simulink model "FMT_G1_ExecutionCore"  (R2026b)
settings: Solver=FixedStepDiscrete  StopTime=2  FixedStep=0.0005
model workspace (MAT data in the model file):
  stop_ticks = 4000
settings Model: Creator=26718  LastModifiedBy=26718

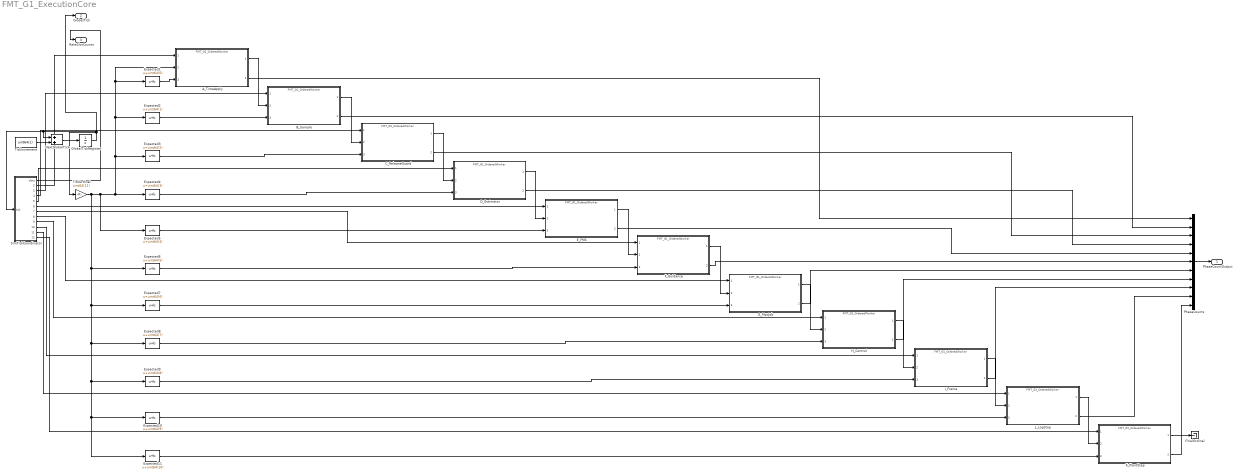
== system FMT_G1_ExecutionCore ==
  A_TimeApply : ModelReference  ModelNameDialog=FMT_G1_OrderedWorker  SimulationMode=Normal  ScheduleRates=on  ModelReferenceVersion=1.2
  B_Sample : ModelReference  ModelNameDialog=FMT_G1_OrderedWorker  SimulationMode=Normal  ScheduleRates=on  ModelReferenceVersion=1.2
  C_ReleaseGuard : ModelReference  ModelNameDialog=FMT_G1_OrderedWorker  SimulationMode=Normal  ScheduleRates=on  ModelReferenceVersion=1.2
  D_Estimator : ModelReference  ModelNameDialog=FMT_G1_OrderedWorker  SimulationMode=Normal  ScheduleRates=on  ModelReferenceVersion=1.2
  E_FMS : ModelReference  ModelNameDialog=FMT_G1_OrderedWorker  SimulationMode=Normal  ScheduleRates=on  ModelReferenceVersion=1.2
  Expected1 : Bias  Bias=uint64(0)  SaturateOnIntegerOverflow=off
  Expected10 : Bias  Bias=uint64(9)  SaturateOnIntegerOverflow=off
  Expected11 : Bias  Bias=uint64(10)  SaturateOnIntegerOverflow=off
  Expected2 : Bias  Bias=uint64(1)  SaturateOnIntegerOverflow=off
  Expected3 : Bias  Bias=uint64(2)  SaturateOnIntegerOverflow=off
  Expected4 : Bias  Bias=uint64(3)  SaturateOnIntegerOverflow=off
  Expected5 : Bias  Bias=uint64(4)  SaturateOnIntegerOverflow=off
  Expected6 : Bias  Bias=uint64(5)  SaturateOnIntegerOverflow=off
  Expected7 : Bias  Bias=uint64(6)  SaturateOnIntegerOverflow=off
  Expected8 : Bias  Bias=uint64(7)  SaturateOnIntegerOverflow=off
  Expected9 : Bias  Bias=uint64(8)  SaturateOnIntegerOverflow=off
  F_Guidance : ModelReference  ModelNameDialog=FMT_G1_OrderedWorker  SimulationMode=Normal  ScheduleRates=on  ModelReferenceVersion=1.2
  FinalOrdinal : Terminator
  G_MpcJob : ModelReference  ModelNameDialog=FMT_G1_OrderedWorker  SimulationMode=Normal  ScheduleRates=on  ModelReferenceVersion=1.2
  GlobalTickRegister : UnitDelay  InitialCondition=uint64(0)  SampleTime=0.0005
  H_Control : ModelReference  ModelNameDialog=FMT_G1_OrderedWorker  SimulationMode=Normal  ScheduleRates=on  ModelReferenceVersion=1.2
  I_Frame : ModelReference  ModelNameDialog=FMT_G1_OrderedWorker  SimulationMode=Normal  ScheduleRates=on  ModelReferenceVersion=1.2
  J_LogStop : ModelReference  ModelNameDialog=FMT_G1_OrderedWorker  SimulationMode=Normal  ScheduleRates=on  ModelReferenceVersion=1.2
  K_PlantStep : ModelReference  ModelNameDialog=FMT_G1_OrderedWorker  SimulationMode=Normal  ScheduleRates=on  ModelReferenceVersion=1.2
  NextGlobalTick : Sum  OutDataTypeStr=uint64
  PhaseCounts : Mux  Inputs=11
  SimTickCoordinator : Stateflow chart  TreatAsAtomicUnit=on
  TickIncrement : Constant  Value=uint64(1)  OutDataTypeStr=uint64
  TickOrdinal : Gain  Gain=uint64(11)  OutDataTypeStr=uint64
  PhaseCountOutput : Outport
  GlobalTick : Outport  Port=2
  RateSlotCounts : Outport  Port=3
  wires:
  K_PlantStep/1 -> FinalOrdinal/1
  K_PlantStep/2 -> PhaseCounts/11
  J_LogStop/1 -> K_PlantStep/2
  Expected11/1 -> K_PlantStep/3
  J_LogStop/2 -> PhaseCounts/10
  I_Frame/1 -> J_LogStop/2
  Expected10/1 -> J_LogStop/3
  I_Frame/2 -> PhaseCounts/9
  H_Control/1 -> I_Frame/2
  Expected9/1 -> I_Frame/3
  H_Control/2 -> PhaseCounts/8
  G_MpcJob/1 -> H_Control/2
  Expected8/1 -> H_Control/3
  G_MpcJob/2 -> PhaseCounts/7
  F_Guidance/1 -> G_MpcJob/2
  Expected7/1 -> G_MpcJob/3
  F_Guidance/2 -> PhaseCounts/6
  E_FMS/1 -> F_Guidance/2
  Expected6/1 -> F_Guidance/3
  E_FMS/2 -> PhaseCounts/5
  D_Estimator/1 -> E_FMS/2
  Expected5/1 -> E_FMS/3
  D_Estimator/2 -> PhaseCounts/4
  C_ReleaseGuard/1 -> D_Estimator/2
  Expected4/1 -> D_Estimator/3
  C_ReleaseGuard/2 -> PhaseCounts/3
  B_Sample/1 -> C_ReleaseGuard/2
  Expected3/1 -> C_ReleaseGuard/3
  B_Sample/2 -> PhaseCounts/2
  A_TimeApply/1 -> B_Sample/2
  Expected2/1 -> B_Sample/3
  A_TimeApply/2 -> PhaseCounts/1
  Expected1/1 -> A_TimeApply/3
  TickOrdinal/1 -> Expected10/1, Expected11/1, Expected9/1, Expected8/1, Expected7/1, Expected6/1, A_TimeApply/2, Expected1/1, Expected2/1, Expected3/1, Expected4/1, Expected5/1
  PhaseCounts/1 -> PhaseCountOutput/1
  SimTickCoordinator/1(slots) -> RateSlotCounts/1
  SimTickCoordinator/2(A_TimeApply()) -> A_TimeApply/1
  SimTickCoordinator/3(B_Sample()) -> B_Sample/1
  SimTickCoordinator/4(C_ReleaseGuard()) -> C_ReleaseGuard/1
  SimTickCoordinator/5(D_Estimator()) -> D_Estimator/1
  SimTickCoordinator/6(E_FMS()) -> E_FMS/1
  SimTickCoordinator/7(F_Guidance()) -> F_Guidance/1
  SimTickCoordinator/8(G_MpcJob()) -> G_MpcJob/1
  SimTickCoordinator/9(H_Control()) -> H_Control/1
  SimTickCoordinator/10(I_Frame()) -> I_Frame/1
  SimTickCoordinator/11(J_LogStop()) -> J_LogStop/1
  SimTickCoordinator/12(K_PlantStep()) -> K_PlantStep/1
  NextGlobalTick/1 -> GlobalTickRegister/1
  TickIncrement/1 -> NextGlobalTick/2
  GlobalTickRegister/1 -> SimTickCoordinator/1(tick), NextGlobalTick/1, GlobalTick/1, TickOrdinal/1

== stateflow chart FMT_G1_ExecutionCore/SimTickCoordinator ==
  settings: updateMethod=DISCRETE  sampleTime=0.0005
  state RUN
    en: slots=zeros(8,1,'uint64');
    if tick < stop_ticks
    slots(1)=slots(1)+uint64(1);
    if rem(tick,uint64(2))==0, slots(2)=slots(2)+uint64(1); end
    if rem(tick,uint64(5))==0, slots(3)=slots(3)+uint64(1); end
    if rem(tick,uint64(20))==0, slots(4)=slots(4)+uint64(1); end
    if rem(tick,uint64(40))==0, slots(5)=slots(5)+uint64(1); end
    if rem(tick,uint64(200))==0, slots(6)=slots(6)+uint64(1); end
    if rem(tick,uint64(2000))==0, slots(7)=slots(7)+uint64(1); slots(8)=slots(8)+uint64(1); end
    A_TimeApply(); B_Sample(); C_ReleaseGuard(); D_Estimator(); E_FMS(); F_Guidance(); G_MpcJob(); H_Control(); I_Frame(); J_LogStop(); K_PlantStep();
    end
    du:
    if tick < stop_ticks
    slots(1)=slots(1)+uint64(1);
    if rem(tick,uint64(2))==0, slots(2)=slots(2)+uint64(1); end
    if rem(tick,uint64(5))==0, slots(3)=slots(3)+uint64(1); end
    if rem(tick,uint64(20))==0, slots(4)=slots(4)+uint64(1); end
    if rem(tick,uint64(40))==0, slots(5)=slots(5)+uint64(1); end
    if rem(tick,uint64(200))==0, slots(6)=slots(6)+uint64(1); end
    if rem(tick,uint64(2000))==0, slots(7)=slots(7)+uint64(1); slots(8)=slots(8)+uint64(1); end
    A_TimeApply(); B_Sample(); C_ReleaseGuard(); D_Estimator(); E_FMS(); F_Guidance(); G_MpcJob(); H_Control(); I_Frame(); J_LogStop(); K_PlantStep();
    end
  (default) -> RUN
  data: slots output uint64; stop_ticks parameter uint64; tick input uint64
  events: A_TimeApply output FUNCTION_CALL_EVENT; B_Sample output FUNCTION_CALL_EVENT; C_ReleaseGuard output FUNCTION_CALL_EVENT; D_Estimator output FUNCTION_CALL_EVENT; E_FMS output FUNCTION_CALL_EVENT; F_Guidance output FUNCTION_CALL_EVENT; G_MpcJob output FUNCTION_CALL_EVENT; H_Control output FUNCTION_CALL_EVENT; I_Frame output FUNCTION_CALL_EVENT; J_LogStop output FUNCTION_CALL_EVENT; K_PlantStep output FUNCTION_CALL_EVENT
